simulink model "RoboCup_ARM"  (R2025b)
settings: Solver=FixedStepAuto  StartTime=0.0  StopTime=12  FixedStep=0.01  RelTol=1e-3
StartFcn:
  | clear attachToRobot
  | clear attachToTool
undefined symbols (not defined in the file or in its folder): gray, Levenberg, Marquardt, q_grip1, Sim3dSensor
libraries: sim3dlib x5, robotcorelib x2, robotmaniplib x2, robotsim3dlib x1, sim3dcameralib x1
settings Model: SimulationMode=accelerator  Creator=Abhishek  LastModifiedBy=ataul

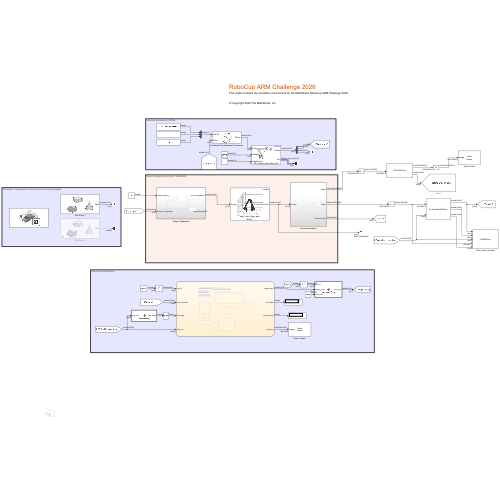
[thumbnail: Simulink's stored preview of the top-level diagram]
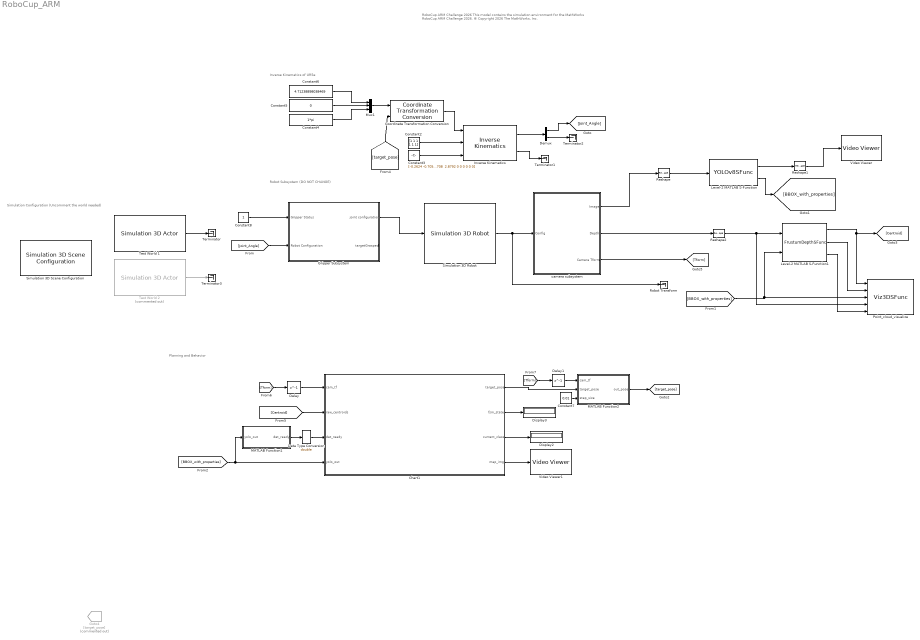
== system RoboCup_ARM ==
  note: Inverse Kinematics of UR5e
  note: Robot Subsystem (DO NOT CHANGE)
  note: Planning and Behavior
  note: Simulation Configuration (Uncomment the world needed)
  note: RoboCup ARM Challenge 2026
      | This model contains the simulation environment for the MathWorks RoboCup ARM Challenge 2026.
      |
      | © Copyright 2026 The MathWorks, Inc.
  Chart1 : Stateflow chart  TreatAsAtomicUnit=on
      settings: PortSchema="{\"entries\":[{\"content\":{\"sides\":[{\"content\":{\"connectorIds\":[\"In1\",\"In3\",\"In2\",\"In4\"]},\"type\":\"ConnectorPlacement.EquallySpacedRectSide\",\"uuid\":\"91c68168-66a8-44f7-9ed5-dcca111e48bd\"},{\"content\":{\"connectorIds\":[\"Out1\",\"Out2\",\"Out3\",\"Out4\"],\"side\":\"RIGHT\"},\"type\":\"ConnectorPlacement.EquallySpacedRectSide\",\"uuid\":\"f9d96617-c5f1-48d2-a824-af271d41434a\"},{\"content\":{\"side\":\"TOP\"},\"type\":\"ConnectorPlacement.EquallySpacedRectSide\",\"uuid\":\"fff7fbd8-46c0-4426-a9b2-1579eb26bf3f\"}]},\"type\":\"ConnectorPlacement.EquallySpacedConnector\",\"uuid\":\"72ef9dc1-c956-4286-9730-cda19fae160c\"}],\"packageUris\":[\"http://schema.mathworks.com/mf0/Connector/R2020b\"],\"version\":\"1.0\"}"
  Constant2 : Constant  Value=[1 1 1 1 1 1]
  Constant3 : Constant  Value="[-0.2624 -0.7054 1.5318 -2.3972 -1.5708  2.8792 0 0 0 0 0 0]"
  Constant4 : Constant  Value=1*pi
  Constant5 : Constant  Value=0
  Constant6 : Constant  Value=4.71238898038469
  Constant7 : Constant  Value=0.01
  Constant8 : Constant
  Coordinate Transformation Conversion : robotcorelib/Coordinate Transformation Conversion  InputRepresentation=Euler Angles  InputEulerSequence=ZYX  ShowTrVecInputPort=on  OutputRepresentation=Homogeneous Transformation  OutputEulerSequence=ZYX  ShowTrVecOutputPort=on  SimulateUsing=Interpreted execution
  Data Type Conversion : DataTypeConversion  OutDataTypeStr=double  SaturateOnIntegerOverflow=off  RndMeth=Floor
  Delay : Delay  DelayLength=1
  Delay1 : Delay  DelayLength=1
  Demux : Demux  Outputs=2
  Display2 : Display
  Display3 : Display
  Goto4 : Goto  Commented=on  GotoTag=target_pose
  Gripper Subsystem : Subsystem
  Inverse Kinematics : robotmaniplib/Inverse Kinematics  RigidBodyTree=rt.robot  EndEffector=robotiq_arg2f_base_link  ShowInfo=on  SolverName=Levenberg-Marquardt  EnforceJointLimits=on  MaxIterations=1500  MaxTime=10  GradientTolerance=1e-3  SolutionTolerance=1e-2  StepTolerance=1e-14  ConstraintTolerance=1e-6  ErrorChangeTolerance=1e-12  UseErrorDamping=on  DampingBias=0.0025  SimulateUsing=Interpreted execution
  Level-2 MATLAB S-Function : M-S-Function  FunctionName=YOLOv8SFunc  Parameters='','others,weight'
  Level-2 MATLAB S-Function1 : M-S-Function  FunctionName=FrustumDepthSFunc  Parameters=1109.0, 1109.0, 640.0, 360.0, 720, 1280
  MATLAB Function1 : MATLAB Function  TreatAsAtomicUnit=on
  MATLAB Function2 : MATLAB Function  TreatAsAtomicUnit=on
  Mux1 : Mux  Inputs=3
  Point_cloud_visualize : M-S-Function  FunctionName=Viz3DSFunc  Parameters=1109.0, 1109.0, 640.0, 360.0, 720, 1280, 'blue_cube,bottle,can,green_cube,marker,others,purple_cube,red_cube,spam,weight'
  Reshape : Reshape
  Reshape1 : Reshape  OutputDimensionality=Customize  OutputDimensions=[720, 1280,3]
  Reshape2 : Reshape
  Robot Transform : Terminator
  Simulation 3D Robot : robotsim3dlib/Simulation 3D Robot  actorInputType=RigidBodyTree Object  RigidBodyTree=rt.robot  ActorName=Robo1  existActorChekBox=on  initialTrans=[0 0 0]  initialRot=[0 0 0]  initialConfig=[-0.2618 -2.1991 1.9722 -1.3963 -1.5882 1.3265 0 0 0 0 0 0]  EndEffector=right_inner_finger_pad  eeOffsetInpChekBox=off  eeTargetTrans=[0 0 0]  eeTargetRot=[0 0 0]  enableRegionGraspChekBox=off  regionGraspInpChekBox=off  eeTargTransDiff=[0.2 0.2 0.2]  eeTargRotDiff=[0 0 0]  enableVisualVisualization=on  enableCollisionVisualization=off  collisionGeomColor=[0 1 0]  collisionGeomTransp=0.1  inpConfEnbVal=on  inpGraspEnbVal=off  inpTransEnbVal=off  outConfEnbVal=on  outGraspEnbVal=off  outTransEnbVal=off  SampleTime=0.01  ActorType=SimulinkVehicle  ID=C  aMode=6  ActorTag=Robo1  Mesh=RigidBodyTree
  Simulation 3D Scene Configuration : sim3dlib/Simulation 3D Scene Configuration  Priority=0  ProjectFormat=Default Scenes  SceneDesc=Empty scene  ProjectName=C:\Program Files\MATLAB\R2025b\toolbox\shared\sim3d_projects\automotive_project_windows\UE\WindowsNoEditor\VehicleSimulation.exe  ScenePath=/Game/Maps/HwStrght  EnableOpenDRIVE=off  vehTagList={'Custom';'Robo1';'Scene Origin';'Sim3dActor1';'Sim3dActor2';'Sim3dActor3';'cameraPlaceHolder'}  vehTag=Scene Origin  AttachedCameraRelativeTranslation=[0 0 0]  FreeCameraDefaultInitialTranslation=[-6, 0, 2]  AttachedCameraRelativeRotation=[0 0 0]  FreeCameraDefaultInitialRotation=[0, -15, 0]  ViewpointName=Custom  FreeCameraInitialTranslation=[0, 0, 0]  ViewpointTranslation=[0 0 0]  FreeCameraInitialRotation=[0, 0, 0]  ViewpointRotation=[0 0 0]  OpVisEn=off  Ts=0.01  EnableWindow=on  EnableRemoteAccess=off  EnableWeather=off  SunAzimuth=90  SunAltitude=40.0  EnableGeospatialSun=off  Latitude=0  Longitude=0  Date=2023-01-01  Time=10:30:00  GeoTimeZone=-5.0  SunDaylightSaving=off  wind=1  clouds=10  EnableVolumetricClouds=off  CloudCoverage=0  CloudAltitude=6  fog=0  rain=0  RaindropsEffect=off  SnowDensity=0  EnableGeospatial=off  TilesetSource=Earth terrain  UseTrueOrigin=off  OriginHeight=200  OriginLatitude=40.744652  OriginLongitude=-73.988864  MapStyle=Aerial  AdditionalAssetIDs=[]  UseAdvancedSunSky=off  SolarTime=11  TimeZone=-5  Day=21  Month=9  Year=2022  UseDaylightSavingTime=on  DSTStartDay=10  DSTStartMonth=3  DSTEndDay=3  DSTEndMonth=11  DSTSwitchHour=2  sensorTag=MainCamera1  sensorId=1  sensorName=MainCamera1  mountLoc=Origin  offsetFlag=off  tmountOffset=[0, 0, 0]  rmountOffset=[0, 0, 0]  HorizontalResolution=1280  VerticalResolution=720  HorizontalFOV=60  mountPoint=[0 0 0]  mountOrientation=[0 0 0]  aMode=5  ID=1  GeoTrigger=Inactive  ViewNameList={'Custom'}  ViewTranslationList={'[0 0 0]'}  ViewRotationList={'[0 0 0]'}
      settings: LibrarySourceBlock=sl3dlib/Simulation 3D/Environment/Simulation 3D Scene Configuration
  Terminator{,1..3} (4 alike) : Terminator
  Test World 1 : sim3dlib/Simulation 3D Actor  Priority=1  ActorName=Sim3dActor1  ParentName=Scene Origin  Operation=Create at setup  InitScriptText=|  SampleTime=-1  Translation=[0 0 0]  Rotation=[0 0 0]  Scale=[1 1 1]  aMode=5  ActorTag=Sim3dActor1  ActorType=Sim3dActor  ID=1
      | % Reserved keywords:
      | % - Actor : handle to this actor object
      | % - World : handle to the world object
      | 
      | % Examples:
      | 
      | % Create a primitive geometry (optional)
      | % createShape(Actor, 'box', [1 1 1]);
      | 
      | % Initialize values (optional)
      | % Actor.Physics = true;
      | % Actor.Color = [1 0 0];
      | Actor.load('example_world.mat')
  Test World 2 : sim3dlib/Simulation 3D Actor  Priority=1  Commented=on  ActorName=Sim3dActor3  ParentName=Scene Origin  Operation=Create at setup  InitScriptText=|  SampleTime=-1  Translation=[0 0 0]  Rotation=[0 0 0]  Scale=[1 1 1]  aMode=5  ActorTag=Sim3dActor3  ActorType=Sim3dActor  ID=3
      | % Reserved keywords:
      | % - Actor : handle to this actor object
      | % - World : handle to the world object
      | 
      | % Examples:
      | 
      | % Create a primitive geometry (optional)
      | % createShape(Actor, 'box', [1 1 1]);
      | 
      | % Initialize values (optional)
      | % Actor.Physics = true;
      | % Actor.Color = [1 0 0];
      | Actor.load('example_world2.mat')
  Video Viewer : VideoViewer  colormapValue=gray(256)  FigPos=[3 1044 1920 933]
  Video Viewer1 : VideoViewer  colormapValue=gray(256)  FigPos=[960 826 418 304]
  camera subsystem : Subsystem
  wires:
  Gripper Subsystem/1(joint configuration) -> Simulation 3D Robot/1
  Simulation 3D Robot/1 -> Robot Transform/1, camera subsystem/1(Config)
  Test World 1/1 -> Terminator/1
  camera subsystem/2(Depth) -> Reshape2/1
  Test World 2/1 -> Terminator3/1
  Coordinate Transformation Conversion/1 -> Inverse Kinematics/1
  Constant2/1 -> Inverse Kinematics/2
  Constant3/1 -> Inverse Kinematics/3
  Inverse Kinematics/2 -> Terminator1/1
  Inverse Kinematics/1 -> Demux/1
  Demux/1 -> [Joint_Angle]
  Demux/2 -> Terminator2/1
  [Joint_Angle] -> Gripper Subsystem/2(Robot Configuration)
  Mux1/1 -> Coordinate Transformation Conversion/1
  Constant5/1 -> Mux1/2
  Constant4/1 -> Mux1/3
  camera subsystem/3(Camera Tform) -> [Tform]
  camera subsystem/1(Image) -> Reshape/1
  Reshape1/1 -> Video Viewer/1
  Reshape/1 -> Level-2 MATLAB S-Function/1
  Level-2 MATLAB S-Function/1 -> Reshape1/1
  Level-2 MATLAB S-Function/2 -> [BBOX_with_properties]
  Reshape2/1 -> Point_cloud_visualize/4, Level-2 MATLAB S-Function1/1
  [BBOX_with_properties] -> Level-2 MATLAB S-Function1/2, Point_cloud_visualize/3
  Level-2 MATLAB S-Function1/1 -> [Centroid], Point_cloud_visualize/1
  Level-2 MATLAB S-Function1/2 -> Point_cloud_visualize/2
  Level-2 MATLAB S-Function1/3 -> Point_cloud_visualize/5
  Constant6/1 -> Mux1/1
  Constant8/1 -> Gripper Subsystem/1(Gripper Status)
  [BBOX_with_properties] -> Chart1/4(yolo_out), MATLAB Function1/1(yolo_out)
  [Centroid] -> Chart1/3(raw_centroids)
  Chart1/1(target_pose) -> MATLAB Function2/2(target_pose)
  Chart1/2(fsm_state) -> Display3/1
  MATLAB Function1/1(det_ready) -> Data Type Conversion/1
  Data Type Conversion/1 -> Chart1/2(det_ready)
  Delay/1 -> Chart1/1(cam_tf)
  [Tform] -> Delay/1
  [target_pose] -> Coordinate Transformation Conversion/2
  MATLAB Function2/1(out_pose) -> [target_pose]
  Constant7/1 -> MATLAB Function2/3(step_size)
  Chart1/3(current_class) -> Display2/1
  [Tform] -> Delay1/1
  Delay1/1 -> MATLAB Function2/1(cam_tf)
  Chart1/4(map_img) -> Video Viewer1/1

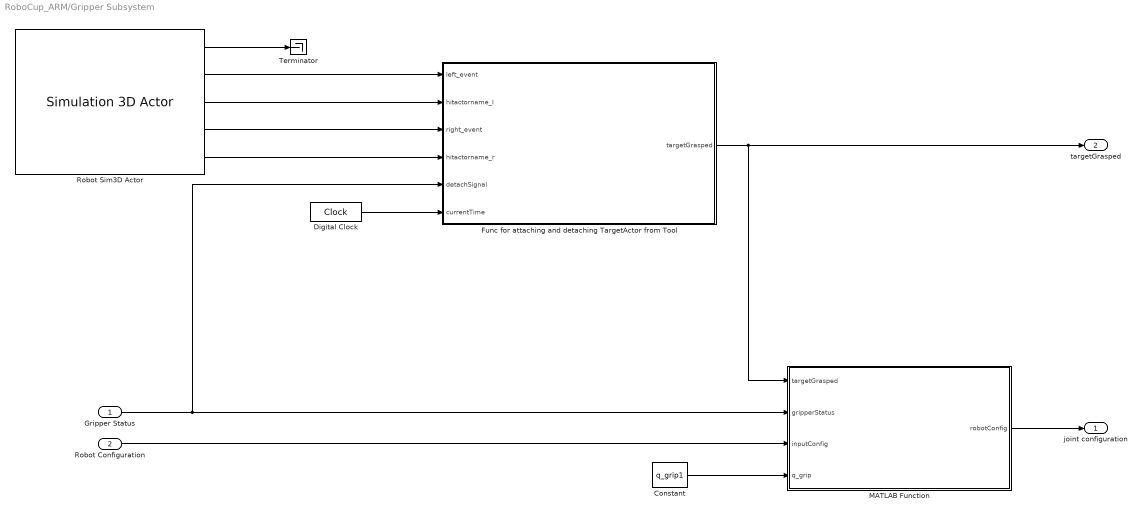
== system RoboCup_ARM/Gripper Subsystem ==
  Gripper Status : Inport
  Robot Configuration : Inport  Port=2
  Constant : Constant  Value=q_grip1
  Digital Clock : DigitalClock
  Func for attaching and detaching TargetActor from Tool : MATLAB Function  TreatAsAtomicUnit=on
  MATLAB Function : MATLAB Function  TreatAsAtomicUnit=on
  Robot Sim3D Actor : sim3dlib/Simulation 3D Actor  Priority=1  ActorName=Sim3dActor2  ParentName=Scene Origin  Operation=Create at setup  InitScriptText=|  SampleTime=-1  Translation=[-0.5 0 1.35]  Rotation=[0 0 0]  Scale=[1 1 1]  EventsText=|  aMode=5  ActorTag=Sim3dActor2  ActorType=Sim3dActor  ID=2
      InitScriptText=|
      | rt = load('ur5e_gripper.mat');
      | robotActor = sim3d.Actor('ActorName', 'Robo1');
      | World.add(robotActor,Actor);
      | 
      | robotActor.load(rt.robot,[1 1 1]);
      | 
      | % finding tool reference 
      | tool1 = World.Actors.left_inner_finger_pad;
      | tool2 = World.Actors.right_inner_finger_pad;
      | tool1.HitEventEnabled = true;
      | tool1.Collisions = true;
      | 
      | tool2.HitEventEnabled = true;
      | tool2.Collisions = true;
      | 
      | %tool1.Physics = true; % somehow this Phsyics dont work
      | % tool1.Color = [10 0 0];
      | tool1.Mobility =  sim3d.utils.MobilityTypes.Movable;
      | 
      | % tool2.Color = [10 0 0];
      | tool2.Mobility =  sim3d.utils.MobilityTypes.Movable;
      | 
      | propagate(World.Actors.('Sim3dActor2'),'Mobility', sim3d.utils.MobilityTypes.Movable);
      | propagate(World.Actors.('Sim3dActor2'),'Shadows',true);
      EventsText=|
      | left_inner_finger_pad.HitEvent          
      | left_inner_finger_pad.HitOtherActorName 
      | right_inner_finger_pad.HitEvent         
      | right_inner_finger_pad.HitOtherActorName
  Terminator : Terminator
  joint configuration : Outport
  targetGrasped : Outport  Port=2
  wires:
  Robot Sim3D Actor/3 -> Func for attaching and detaching TargetActor from Tool/2(hitactorname_l)
  Robot Sim3D Actor/2 -> Func for attaching and detaching TargetActor from Tool/1(left_event)
  Robot Sim3D Actor/4 -> Func for attaching and detaching TargetActor from Tool/3(right_event)
  Robot Sim3D Actor/5 -> Func for attaching and detaching TargetActor from Tool/4(hitactorname_r)
  Digital Clock/1 -> Func for attaching and detaching TargetActor from Tool/6(currentTime)
  Gripper Status/1 -> Func for attaching and detaching TargetActor from Tool/5(detachSignal), MATLAB Function/2(gripperStatus)
  Robot Configuration/1 -> MATLAB Function/3(inputConfig)
  Func for attaching and detaching TargetActor from Tool/1(targetGrasped) -> MATLAB Function/1(targetGrasped), targetGrasped/1
  Constant/1 -> MATLAB Function/4(q_grip)
  MATLAB Function/1(robotConfig) -> joint configuration/1
  Robot Sim3D Actor/1 -> Terminator/1

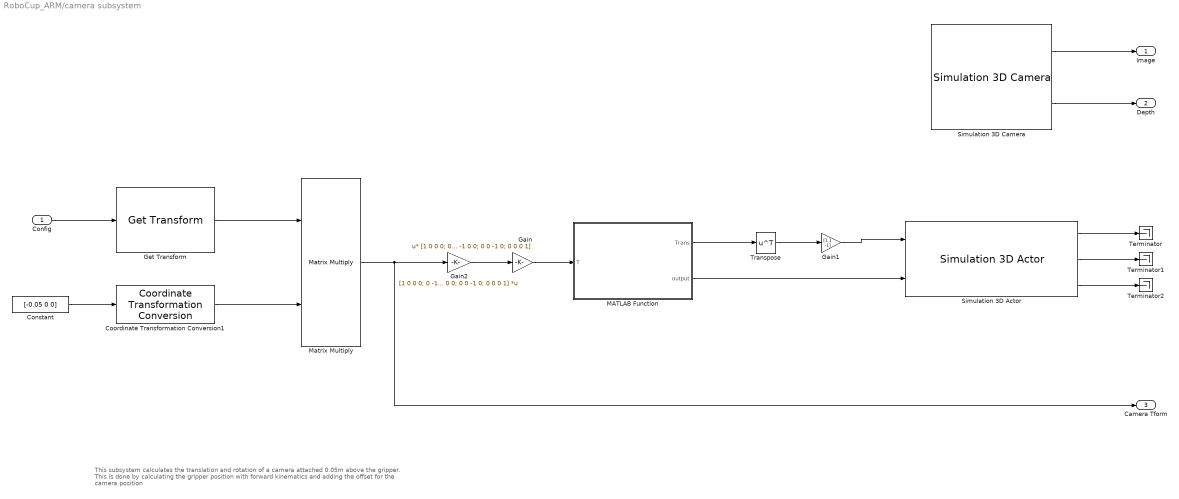
== system RoboCup_ARM/camera subsystem ==
  note: This subsystem calculates the translation and rotation of a camera attached 0.05m above the gripper. This is done by calculating the gripper position with forward kinematics and adding the offset for the camera position
  Config : Inport
  Constant : Constant  Value=[-0.05 0 0]
  Coordinate Transformation Conversion1 : robotcorelib/Coordinate Transformation Conversion  InputRepresentation=Translation Vector  InputEulerSequence=ZYX  ShowTrVecInputPort=on  OutputRepresentation=Homogeneous Transformation  OutputEulerSequence=ZYX  ShowTrVecOutputPort=on  SimulateUsing=Interpreted execution
      settings: LibrarySourceBlock=navlib/Utilities/Coordinate Transformation Conversion
  Gain : Gain  Gain=[1 0 0 0; 0 -1 0 0; 0 0 -1 0; 0 0 0 1]  Multiplication=Matrix(u*K)
  Gain1 : Gain  Gain=[1 1 -1]
  Gain2 : Gain  Gain=[1 0 0 0; 0 -1 0 0; 0 0 -1 0; 0 0 0 1]  Multiplication=Matrix(K*u)
  Get Transform : robotmaniplib/Get Transform  RigidBodyTree=rt.robot  SourceBody=robotiq_arg2f_base_link  TargetBody=base_link  SimulateUsing=Interpreted execution
  MATLAB Function : MATLAB Function  TreatAsAtomicUnit=on
  Matrix Multiply : Product  Multiplication=Matrix(*)
  Simulation 3D Actor : sim3dlib/Simulation 3D Actor  Priority=1  ActorName=cameraPlaceHolder  ParentName=Robo1  Operation=Create at setup  InitScriptText=|  SampleTime=-1  Translation=[0.05 0 0]  Rotation=[0 0 0]  Scale=[1 1 1]  InputsText=cameraPlaceHolder.Translation cameraPlaceHolder.Rotation  OutputsText=cameraPlaceHolder.Translation cameraPlaceHolder.Rotation  aMode=5  ActorTag=cameraPlaceHolder  ActorType=Sim3dActor  ID=C
      | Actor.createShape('box', [0.02 0.04 0.06]);
      | Actor.Mobility=sim3d.utils.MobilityTypes.Movable;
      | Actor.Color=[1 0 0];
      | Actor.Translation=[0.05, 0, 0];
      | Actor.Rotation = [0, 0, 0];
      | Actor.ConstantAttributes=false;
      | Actor.Mass = 1;
      | Actor.Transparency = 0;
      | Actor.Shininess = 0;
  Simulation 3D Camera : sim3dcameralib/Simulation 3D Camera  Priority=1  sensorTag=Sim3dSensor�  sensorId=1  sensorName=Sim3dSensor1  vehTagList={'Robo1';'Scene Origin';'Sim3dActor1';'Sim3dActor2';'Sim3dActor3';'cameraPlaceHolder'}  vehTag=cameraPlaceHolder  CoordinateSystem=ISO8855  mountLoc=Origin  offsetFlag=on  tmountOffset=[0 0 0]  extTmount=off  rmountOffset=[0, -90, 0]  extRmount=off  FocalLength=[1109, 1109]  OpticalCenter=[640, 360]  ImageSize=[720, 1280]  RadialDistortion=[0, 0]  TangentialDistortion=[0, 0]  SensorSkew=0  VisualizeFieldOfView=on  FieldOfViewRange=61  DepthOutportEnabled=on  SemanticOutportEnabled=off  TransformOutportEnabled=off  SampleTime=0.01  mountPoint=[0 0 0]  mountOrientation=[0 -90 0]  aMode=5  ID=1
      settings: LibrarySourceBlock=sl3dlib/Simulation 3D/Sensors/Simulation 3D Camera
  Terminator : Terminator
  Terminator1 : Terminator
  Terminator2 : Terminator
  Transpose : Math  Operator=transpose
  Image : Outport
  Depth : Outport  Port=2
  Camera Tform : Outport  Port=3
  wires:
  MATLAB Function/1(Trans) -> Transpose/1
  Coordinate Transformation Conversion1/1 -> Matrix Multiply/2
  Simulation 3D Actor/2 -> Terminator1/1
  Transpose/1 -> Gain1/1
  Simulation 3D Camera/2 -> Depth/1
  Simulation 3D Actor/1 -> Terminator/1
  Gain/1 -> MATLAB Function/1(T)
  Simulation 3D Actor/3 -> Terminator2/1
  MATLAB Function/2(output) -> Simulation 3D Actor/2
  Matrix Multiply/1 -> Gain2/1, Camera Tform/1
  Gain1/1 -> Simulation 3D Actor/1
  Get Transform/1 -> Matrix Multiply/1
  Simulation 3D Camera/1 -> Image/1
  Gain2/1 -> Gain/1
  Constant/1 -> Coordinate Transformation Conversion1/1
  Config/1 -> Get Transform/1

== matlab function RoboCup_ARM/MATLAB Function2 ==
  data: cam_tf input; target_pose input; out_pose output; step_size input
function out_pose = interpolatePose(cam_tf, target_pose, step_size)
    persistent current_pose;
    if isempty(current_pose)
        current_pose = target_pose;
    end
    
    curr_pos = cam_tf(1:3,4);
    dist = norm(curr_pos(1:2) - target_pose(1:2));
    
    if dist > step_size
        diff = target_pose - current_pose;
        next_pose = current_pose + step_size * diff/norm(diff);
        
        % Dead zone check
        if sqrt(next_pose(1)^2 + next_pose(2)^2) > 0.3
            current_pose = next_pose;
        end
    else
        current_pose = target_pose;
    end
    
    out_pose = current_pose;
end

== stateflow chart RoboCup_ARM/Chart1 ==
  state Centroid_dwell
    entry:
    fsm_state = 5;
    for i = pick_idx:queue_size-1
    pick_queue(i,:) = pick_queue(i+1,:);
    end
    pick_queue(queue_size,:) = zeros(1,4);
    queue_size = queue_size - 1;
    map_img = updateOccupancyMap(map_img, pick_queue(pick_idx,1), pick_queue(pick_idx,2), pick_queue(pick_idx,4), 1);
  state Done
    entry:
    fsm_state = 6;
  state Init
    entry:
    fsm_state = 0;
    [scanX, scanY, N] = buildScanPath();
    scan_idx   = 1;
    scan_z     = 0.55;
    tol        = 0.05;
    pick_queue = zeros(20,4);
    queue_size = 0;
    pick_idx   = 0;
    log_count  = 0;
    target_pose = [scanX(1); scanY(1); scan_z];
    map_img = zeros(24, 15, 3, 'uint8');
  state Centroid_move
    entry:
    fsm_state = 4;
    pick_idx = findNearest(cam_tf(1:3,4), pick_queue, queue_size);
    if pick_idx > 0
    target_pose = [pick_queue(pick_idx,1); pick_queue(pick_idx,2); scan_z];
    current_class = pick_queue(pick_idx,4);
    end
  state Home_wait
    entry:
    fsm_state = 1;
    target_pose = [scanX(1); scanY(1); scan_z];
  state Scan_Dwell
    entry:
    fsm_state = 3;
    if det_ready == 1
    for i = 1:20
    nc = raw_centroids(i,:);
    if norm(nc(1:3)) < 0.001, continue; end
    if sqrt(nc(1)^2 + nc(2)^2) < 0.3, continue; end
    if queue_size < 20
    queue_size = queue_size + 1;
    pick_queue(queue_size,1:3) = nc;
    pick_queue(queue_size,4) = yolo_out(i,6);
    map_img = updateOccupancyMap(map_img, nc(1), nc(2), yolo_out(i,6), 1);
    end
    end
    end
    map_img = updateOccupancyMap(map_img, scanX(scan_idx), scanY(scan_idx), 0, 0);
    scan_idx = scan_idx + 1;
  state Scan_Move
    entry:
    fsm_state = 2;
    target_pose = [scanX(scan_idx); scanY(scan_idx); scan_z];
  (default) -> Init
  Centroid_dwell -> Done [order 2] : [queue_size == 0]
  Centroid_dwell -> Centroid_move [order 1] : [queue_size > 0]
  Centroid_move -> Centroid_dwell [order 1] : [isAtTarget(cam_tf, target_pose, tol) || after(0.2, sec)]
  Centroid_move -> Done [order 2] : [pick_idx == -1]
  Init -> Home_wait
  Scan_Dwell -> Centroid_move [order 1] : [scan_idx > N]
  Home_wait -> Scan_Move : after(0.1, sec)
  Scan_Move -> Scan_Dwell : [isAtTarget(cam_tf, target_pose, tol) || after(0.2, sec)]
  Scan_Dwell -> Scan_Move [order 2] : [scan_idx <= N]
  data: cam_tf_in function_input; target_pose_in function_input; tol_in function_input; reached function_output; map_img function_input; x function_input; y function_input; class_id function_input; mode function_input; map_img function_output; pos function_input; queue function_input; qsize function_input; idx function_output; sX function_output; sY function_output; N function_output; cam_tf input double size=[4,4]; det_ready input double size=1; raw_centroids input double size=[20,3]; target_pose output double size=[3,1]; fsm_state output double size=1; scanX local double size=[1,24]; scanY local double size=[1,24]; N local double size=1; scan_idx local double size=1; scan_z local double size=1; tol local double size=1; pick_queue local double size=[20,4]; queue_size local double size=1; pick_idx local double size=1; log_count local double size=1; i local size=1; nc local size=[1,3]; yolo_out input size=[20,6]; current_class output size=1; map_img output
  function reached = isAtTarget(cam_tf_in, target_pose_in, tol_in):
    | function reached = isAtTarget(cam_tf_in, target_pose_in, tol_in)
    |     cam_offset = [0; 0; 0];
    |     curr_pos = cam_tf_in(1:3,4) - cam_offset;
    |     dist = sqrt((curr_pos(1) - target_pose_in(1))^2 + (curr_pos(2) - target_pose_in(2))^2);
    |     reached = dist <= tol_in;
    | end
  function map_img = updateOccupancyMap(map_img, x, y, class_id, mode):
    | function map_img = updateOccupancyMap(map_img, x, y, class_id, mode)
    |     x_min = 0.10; x_max = 0.85;
    |     y_min = -0.60; y_max = 0.60;
    |     cols = 15; rows = 24;
    | 
    |     colors = uint8([
    |           0, 114, 189;
    |           0, 190, 190;
    |         217, 120,   0;
    |          50, 168,  82;
    |         162,   0, 162;
    |           0,   0,   0;
    |         102,   0, 204;
    |         220,   0,   0;
    |         204, 180,   0;
    |     ]);
    | 
    |     col = round(1 + (x - x_min)/(x_max - x_min) * (cols-1));
    |     row = round(1 + (y - y_min)/(y_max - y_min) * (rows-1));
    |     col = max(1, min(cols, col));
    |     row = max(1, min(rows, row));
    | 
    |     if mode == 0
    |         map_img(row, col, 1) = 128;
    |         map_img(row, col, 2) = 128;
    |         map_img(row, col, 3) = 128;
    |     elseif mode == 1 && ~ismember(class_id, [5, 9])
    |         map_img(row, col, 1) = colors(class_id+1, 1);
    |         map_img(row, col, 2) = colors(class_id+1, 2);
    |         map_img(row, col, 3) = colors(class_id+1, 3);
    |     end
    | end
  function idx = findNearest(pos, queue, qsize):
    | function idx = findNearest(pos, queue, qsize)
    |     idx = -1; best = inf;
    |     SKIP = [5,7,9];
    |     for i = 1:qsize
    |         cx = queue(i,1); cy = queue(i,2);
    |         if sqrt(cx^2+cy^2) < 0.3, continue; end
    |         if ismember(queue(i,4), SKIP), continue; end
    |         d = norm(queue(i,1:3) - pos(:)');
    |         if d < best, best = d; idx = i; end
    |     end
    | end
  function [sX, sY, N] = buildScanPath:
    | function [sX, sY, N] = buildScanPath()
    |     sX = zeros(1,24); sY = zeros(1,24); N = 0;
    |     xVals = [0.10, 0.35, 0.60, 0.85];
    |     yVals = [-0.6, -0.35, -0.10, 0.15, 0.40, 0.6];
    |     allX = zeros(1,24); allY = zeros(1,24); k = 0;
    |     for row = 1:6
    |         if mod(row,2)==1, rowX = xVals;
    |         else, rowX = [0.85,0.60,0.35,0.10]; end
    |         for col = 1:4
    |             k = k+1; allX(k) = rowX(col); allY(k) = yVals(row);
    |         end
    |     end
    |     count = 0;
    |     for i = 1:24
    |         if sqrt(allX(i)^2 + allY(i)^2) > 0.3
    |             count = count+1;
    |             sX(count) = allX(i);
    |             sY(count) = allY(i);
    |         end
    |     end
    |     N = count;
    | end

== matlab function RoboCup_ARM/MATLAB Function1 ==
  data: yolo_out input; det_ready output
function det_ready = calcDetReady(yolo_out)
    % Ready if at least one row has confidence > 0.5
    det_ready = any(yolo_out(:,5) > 0.5);
end

== matlab function RoboCup_ARM/Gripper Subsystem/MATLAB Function ==
  data: targetGrasped input; robotConfig output; gripperStatus input; inputConfig input; q_grip input
function robotConfig = appendGripper(targetGrasped, gripperStatus, inputConfig, q_grip)

persistent index
if isempty(index)
    index = 1;
end

% Open gripper
if ~gripperStatus
    openConfig = [0 0 0 0 0 0]';
    robotConfig = [inputConfig; openConfig]';
    index = 1;
else
    if index > size(q_grip, 2)
        robotConfig = [inputConfig; q_grip(:, index-1)]';
        index = 1;
    elseif targetGrasped
        robotConfig = [inputConfig; q_grip(:, index)]';
    else
        robotConfig = [inputConfig; q_grip(:, index)]';
        index = index + 1;
    end
end

== matlab function RoboCup_ARM/Gripper Subsystem/Func for attaching and detaching TargetActor from Tool ==
  data: left_event input; targetGrasped output; hitactorname_l input; right_event input; hitactorname_r input; detachSignal input; currentTime input
 function targetGrasped = attachToRobot(left_event, hitactorname_l, right_event, hitactorname_r, detachSignal, currentTime)
    
    persistent l_time r_time grasped;
    if isempty(l_time)
        l_time = 0;
    end

    if isempty(r_time)
        r_time = 1;
    end

    if left_event
        l_time = currentTime;
    end

    if right_event
        r_time = currentTime;
    end
    
    if isempty(grasped)
        grasped = 0;
    end

    targetGrasped = grasped;

    coder.extrinsic('attachToTool');

    if abs(l_time - r_time) < 0.5 || ~detachSignal
        grasped = attachToTool(hitactorname_l, hitactorname_r,detachSignal);
        targetGrasped = grasped;
    end
end

== matlab function RoboCup_ARM/camera subsystem/MATLAB Function ==
  data: T input; Trans output; output output
function [Trans, output] = rotm2fixedZYX(T)
    R = T(1:3,1:3);
    Trans = T(1:3,4);
    if abs(R(3,1)) < 1
        pitch = -asin(R(3,1));
        roll  = atan2(R(3,2)/cos(pitch), R(3,3)/cos(pitch));
        yaw   = atan2(R(2,1)/cos(pitch), R(1,1)/cos(pitch));
    else
        % Gimbal lock
        if R(3,1) <= -1
            pitch = pi/2;
        else
            pitch = -pi/2;
        end
        yaw = 0;
        roll = atan2(-R(1,2), R(1,3));
    end
    output = [roll, pitch, yaw];
end
